simulink model "dummy_system"  (R2019a)
settings: Solver=VariableStepAuto  StartTime=0.0  StopTime=10.0  MaxStep=0.2  RelTol=1e-3
values from neighbouring files (symbols this model uses):
  A = [-0.98, 0; 0, -0.9]    [passing_data_training.m]
  B = [1 0; 0,0]    [passing_data_training.m]
  C = [1,0;0,1]    [passing_data_training.m]
  D = [0,0;0,0]    [passing_data_training.m]
  X0 = [pi;2]    [passing_data_training.m]
libraries: simulink x1
settings Model: Creator=joakira  LastModifiedBy=joakira

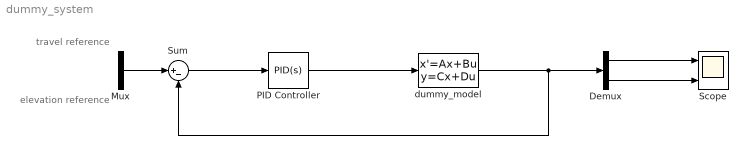
== system dummy_system ==
  note: elevation reference
  note: travel reference
  Demux : Demux  Outputs=2
  Mux : Mux  Inputs=2
  PID Controller : simulink/Continuous/PID Controller  Controller=PID  Form=Parallel  TimeDomain=Continuous-time  SampleTime=-1  IntegratorMethod=Forward Euler  FilterMethod=Forward Euler  ControllerParametersSource=internal  P=10  I=20  D=0  UseFilter=on  N=100  TunerSelectOption=Transfer Function Based (PID Tuner App)  InitialConditionSource=internal  InitialConditionForIntegrator=0  InitialConditionForFilter=0  DifferentiatorICPrevScaledInput=0  ExternalReset=none  TrackingMode=off  Kt=1  LimitOutput=off  UpperSaturationLimit=inf  LowerSaturationLimit=-inf  LinearizeAsGain=on  AntiWindupMode=none  Kb=1  POutMin=[]  POutMax=[]  IOutMin=[]  IOutMax=[]  DOutMin=[]  DOutMax=[]  NOutMin=[]  NOutMax=[]  SumOutMin=[]  SumOutMax=[]  SaturationOutMin=[]  SaturationOutMax=[]  PParamMin=[]  PParamMax=[]  IParamMin=[]  IParamMax=[]  DParamMin=[]  DParamMax=[]  NParamMin=[]  NParamMax=[]  KbParamMin=[]  KbParamMax=[]  KtParamMin=[]  KtParamMax=[]  KbOutMin=[]  KbOutMax=[]  KtOutMin=[]  KtOutMax=[]  IntegratorOutMin=[]  IntegratorOutMax=[]  FilterOutMin=[]  FilterOutMax=[]  SumI1OutMin=[]  SumI1OutMax=[]  SumI2OutMin=[]  SumI2OutMax=[]  SumI3OutMin=[]  SumI3OutMax=[]  SumI4OutMin=[]  SumI4OutMax=[]  SumDOutMin=[]  SumDOutMax=[]  DifferentiatorOutMin=[]  DifferentiatorOutMax=[]  FilterDiffOutCoefMin=[]  FilterDiffOutCoefMax=[]  ReciprocalOutMin=[]  ReciprocalOutMax=[]  SumDenOutMin=[]  SumDenOutMax=[]  SumNumOutMin=[]  SumNumOutMax=[]  DivideOutMin=[]  DivideOutMax=[]  IntegratorContinuousStateAttributes=''  IntegratorStateMustResolveToSignalObject=off  IntegratorRTWStateStorageClass=Auto  FilterContinuousStateAttributes=''  FilterStateMustResolveToSignalObject=off  FilterRTWStateStorageClass=Auto  ParallelPVariant=InternalParameters  IdealPVariant=Disabled  IVariant=InternalParameters  DVariant=InternalParameters  IntegratorVariant=Continuous  SatVariant=Disabled  AWVariant=Passthrough  PCopyVariant=Disabled  TRVariant=Disabled  FdbkBlocksVariant=Forward  IdealPFdbkVariant=Disabled  SatFdbkVariant=Disabled  DerivativeFilterVariant=ContFilter  NVariant=InternalParameters  NCopyVariant=Disabled  FilterICVariant=InternalICsFilter  IntegratorICVariant=InternalICs  ExternalResetVariant=Disabled  TRSumVariant=Passthrough  SumFdbkVariant=Disabled  SumVariant=Sum_PID
  Scope : Scope  NumInputPorts=2
  Sum : Sum  Inputs=|+-
  dummy_model : StateSpace  A=A  B=B  C=C  D=D  InitialCondition=X0
  wires:
  dummy_model/1 -> Demux/1, Sum/2
  Sum/1 -> PID Controller/1
  PID Controller/1 -> dummy_model/1
  Demux/1 -> Scope/1
  Demux/2 -> Scope/2
  Mux/1 -> Sum/1
